simulink model "ADCS_FSM_test"  (R2025b)
settings: Solver=FixedStepDiscrete  StartTime=0.0  StopTime=10  FixedStep=0.1  RelTol=1e-3
settings Model: Creator=ADMIN  LastModifiedBy=ADMIN
settings DataIOCC: ExternalInput=ds  LoadExternalInput=on

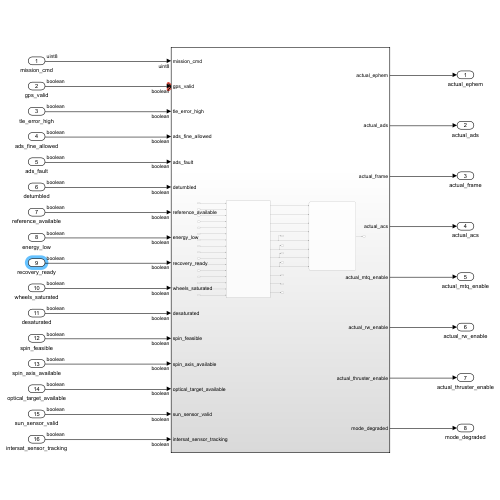
[thumbnail: Simulink's stored preview of the top-level diagram]
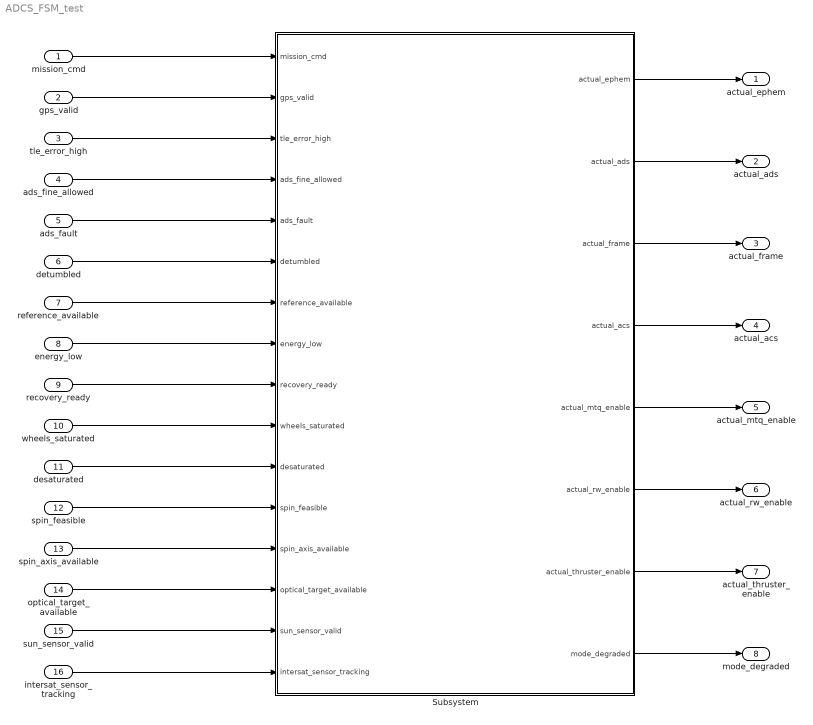
== system ADCS_FSM_test ==
  mission_cmd : Inport  OutDataTypeStr=uint8  PortDimensions=1
  gps_valid : Inport  Port=2  OutDataTypeStr=boolean  PortDimensions=1
  tle_error_high : Inport  Port=3  OutDataTypeStr=boolean  PortDimensions=1
  ads_fine_allowed : Inport  Port=4  OutDataTypeStr=boolean  PortDimensions=1
  ads_fault : Inport  Port=5  OutDataTypeStr=boolean  PortDimensions=1
  detumbled : Inport  Port=6  OutDataTypeStr=boolean  PortDimensions=1
  reference_available : Inport  Port=7  OutDataTypeStr=boolean  PortDimensions=1
  energy_low : Inport  Port=8  OutDataTypeStr=boolean  PortDimensions=1
  recovery_ready : Inport  Port=9  OutDataTypeStr=boolean  PortDimensions=1
  wheels_saturated : Inport  Port=10  OutDataTypeStr=boolean  PortDimensions=1
  desaturated : Inport  Port=11  OutDataTypeStr=boolean  PortDimensions=1
  spin_feasible : Inport  Port=12  OutDataTypeStr=boolean  PortDimensions=1
  spin_axis_available : Inport  Port=13  OutDataTypeStr=boolean  PortDimensions=1
  optical_target_available : Inport  Port=14  OutDataTypeStr=boolean  PortDimensions=1
  sun_sensor_valid : Inport  Port=15  OutDataTypeStr=boolean  PortDimensions=1
  intersat_sensor_tracking : Inport  Port=16  OutDataTypeStr=boolean  PortDimensions=1
  Subsystem : Subsystem
  actual_ephem : Outport
  actual_ads : Outport  Port=2
  actual_frame : Outport  Port=3
  actual_acs : Outport  Port=4
  actual_mtq_enable : Outport  Port=5
  actual_rw_enable : Outport  Port=6
  actual_thruster_enable : Outport  Port=7
  mode_degraded : Outport  Port=8
  wires:
  mission_cmd/1 -> Subsystem/1(mission_cmd)
  tle_error_high/1 -> Subsystem/3(tle_error_high)
  ads_fine_allowed/1 -> Subsystem/4(ads_fine_allowed)
  ads_fault/1 -> Subsystem/5(ads_fault)
  wheels_saturated/1 -> Subsystem/10(wheels_saturated)
  Subsystem/1(actual_ephem) -> actual_ephem/1
  Subsystem/8(mode_degraded) -> mode_degraded/1
  Subsystem/2(actual_ads) -> actual_ads/1
  Subsystem/3(actual_frame) -> actual_frame/1
  Subsystem/4(actual_acs) -> actual_acs/1
  Subsystem/5(actual_mtq_enable) -> actual_mtq_enable/1
  Subsystem/6(actual_rw_enable) -> actual_rw_enable/1
  Subsystem/7(actual_thruster_enable) -> actual_thruster_enable/1
  recovery_ready/1 -> Subsystem/9(recovery_ready)
  spin_feasible/1 -> Subsystem/12(spin_feasible)
  spin_axis_available/1 -> Subsystem/13(spin_axis_available)
  sun_sensor_valid/1 -> Subsystem/15(sun_sensor_valid)
  gps_valid/1 -> Subsystem/2(gps_valid)
  detumbled/1 -> Subsystem/6(detumbled)
  reference_available/1 -> Subsystem/7(reference_available)
  energy_low/1 -> Subsystem/8(energy_low)
  desaturated/1 -> Subsystem/11(desaturated)
  optical_target_available/1 -> Subsystem/14(optical_target_available)
  intersat_sensor_tracking/1 -> Subsystem/16(intersat_sensor_tracking)

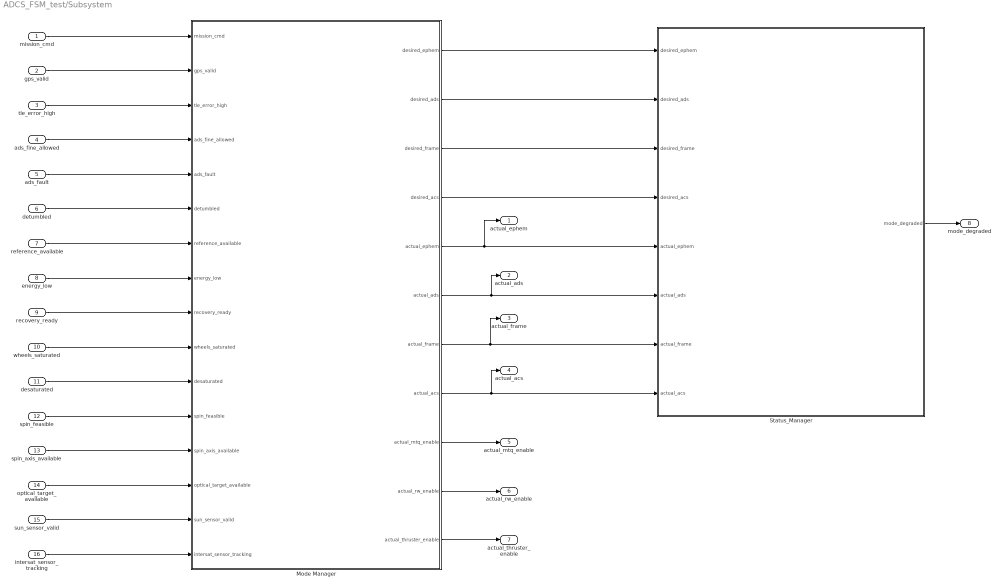
== system ADCS_FSM_test/Subsystem ==
  mission_cmd : Inport
  gps_valid : Inport  Port=2
  tle_error_high : Inport  Port=3
  ads_fine_allowed : Inport  Port=4
  ads_fault : Inport  Port=5
  detumbled : Inport  Port=6
  reference_available : Inport  Port=7
  energy_low : Inport  Port=8
  recovery_ready : Inport  Port=9
  wheels_saturated : Inport  Port=10
  desaturated : Inport  Port=11
  spin_feasible : Inport  Port=12
  spin_axis_available : Inport  Port=13
  optical_target_available : Inport  Port=14
  sun_sensor_valid : Inport  Port=15
  intersat_sensor_tracking : Inport  Port=16
  Mode Manager : Subsystem
  Status_Manager : Stateflow chart  TreatAsAtomicUnit=on
  actual_ephem : Outport
  actual_ads : Outport  Port=2
  actual_frame : Outport  Port=3
  actual_acs : Outport  Port=4
  actual_mtq_enable : Outport  Port=5
  actual_rw_enable : Outport  Port=6
  actual_thruster_enable : Outport  Port=7
  mode_degraded : Outport  Port=8
  wires:
  recovery_ready/1 -> Mode Manager/9(recovery_ready)
  Mode Manager/9(actual_mtq_enable) -> actual_mtq_enable/1
  Mode Manager/10(actual_rw_enable) -> actual_rw_enable/1
  Mode Manager/2(desired_ads) -> Status_Manager/2(desired_ads)
  Mode Manager/8(actual_acs) -> Status_Manager/8(actual_acs), actual_acs/1
  Mode Manager/1(desired_ephem) -> Status_Manager/1(desired_ephem)
  Mode Manager/5(actual_ephem) -> Status_Manager/5(actual_ephem), actual_ephem/1
  Mode Manager/6(actual_ads) -> Status_Manager/6(actual_ads), actual_ads/1
  Mode Manager/7(actual_frame) -> Status_Manager/7(actual_frame), actual_frame/1
  Mode Manager/3(desired_frame) -> Status_Manager/3(desired_frame)
  Mode Manager/4(desired_acs) -> Status_Manager/4(desired_acs)
  reference_available/1 -> Mode Manager/7(reference_available)
  mission_cmd/1 -> Mode Manager/1(mission_cmd)
  ads_fault/1 -> Mode Manager/5(ads_fault)
  ads_fine_allowed/1 -> Mode Manager/4(ads_fine_allowed)
  Mode Manager/11(actual_thruster_enable) -> actual_thruster_enable/1
  wheels_saturated/1 -> Mode Manager/10(wheels_saturated)
  optical_target_available/1 -> Mode Manager/14(optical_target_available)
  detumbled/1 -> Mode Manager/6(detumbled)
  intersat_sensor_tracking/1 -> Mode Manager/16(intersat_sensor_tracking)
  desaturated/1 -> Mode Manager/11(desaturated)
  spin_feasible/1 -> Mode Manager/12(spin_feasible)
  tle_error_high/1 -> Mode Manager/3(tle_error_high)
  energy_low/1 -> Mode Manager/8(energy_low)
  Status_Manager/1(mode_degraded) -> mode_degraded/1
  spin_axis_available/1 -> Mode Manager/13(spin_axis_available)
  sun_sensor_valid/1 -> Mode Manager/15(sun_sensor_valid)
  gps_valid/1 -> Mode Manager/2(gps_valid)

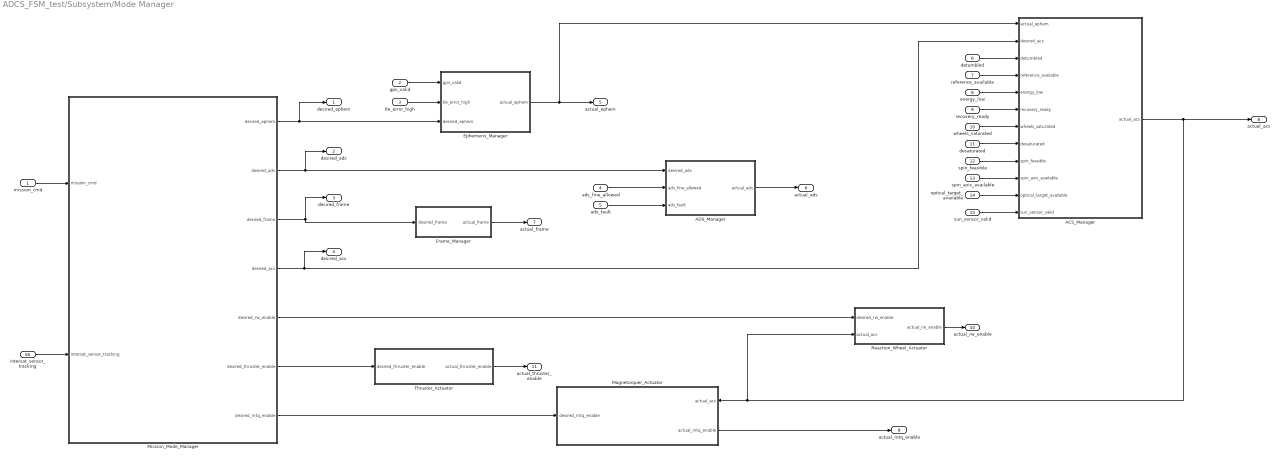
== system ADCS_FSM_test/Subsystem/Mode Manager ==
  mission_cmd : Inport  OutDataTypeStr=uint8  PortDimensions=1
  gps_valid : Inport  Port=2  OutDataTypeStr=boolean  PortDimensions=1
  tle_error_high : Inport  Port=3  OutDataTypeStr=boolean  PortDimensions=1
  ads_fine_allowed : Inport  Port=4  OutDataTypeStr=boolean  PortDimensions=1
  ads_fault : Inport  Port=5  OutDataTypeStr=boolean  PortDimensions=1
  detumbled : Inport  Port=6  OutDataTypeStr=boolean  PortDimensions=1
  reference_available : Inport  Port=7  OutDataTypeStr=boolean  PortDimensions=1
  energy_low : Inport  Port=8  OutDataTypeStr=boolean  PortDimensions=1
  recovery_ready : Inport  Port=9  OutDataTypeStr=boolean  PortDimensions=1
  wheels_saturated : Inport  Port=10  OutDataTypeStr=boolean  PortDimensions=1
  desaturated : Inport  Port=11  OutDataTypeStr=boolean  PortDimensions=1
  spin_feasible : Inport  Port=12  OutDataTypeStr=boolean  PortDimensions=1
  spin_axis_available : Inport  Port=13  OutDataTypeStr=boolean  PortDimensions=1
  optical_target_available : Inport  Port=14  OutDataTypeStr=boolean  PortDimensions=1
  sun_sensor_valid : Inport  Port=15  OutDataTypeStr=boolean  PortDimensions=1
  intersat_sensor_tracking : Inport  Port=16  OutDataTypeStr=boolean  PortDimensions=1
  ACS_Manager : Stateflow chart  TreatAsAtomicUnit=on
      settings: PortSchema="{\"entries\":[{\"content\":{\"sides\":[{\"content\":{\"connectorIds\":[\"In2\",\"In1\",\"In3\",\"In4\",\"In5\",\"In6\",\"In7\",\"In8\",\"In9\",\"In10\",\"In11\",\"In12\"]},\"type\":\"ConnectorPlacement.EquallySpacedRectSide\",\"uuid\":\"c64f5ed7-7a07-4761-a251-d625087249f8\"},{\"content\":{\"connectorIds\":[\"Out1\"],\"side\":\"RIGHT\"},\"type\":\"ConnectorPlacement.EquallySpacedRectSide\",\"uuid\":\"ff17dfa7-5a32-4799-bec0-131df3b46d45\"},{\"content\":{\"side\":\"TOP\"},\"type\":\"ConnectorPlacement.EquallySpacedRectSide\",\"uuid\":\"acaf274e-12ec-4fab-ab7e-ad580afcef6e\"}]},\"type\":\"ConnectorPlacement.EquallySpacedConnector\",\"uuid\":\"7d19de63-b993-417e-b6e9-9dc888da130b\"}],\"packageUris\":[\"http://schema.mathworks.com/mf0/Connector/R2020b\"],\"version\":\"1.0\"}"
  ADS_Manager : Stateflow chart  TreatAsAtomicUnit=on
  Ephemeris_Manager : Stateflow chart  TreatAsAtomicUnit=on
      settings: PortSchema="{\"entries\":[{\"content\":{\"sides\":[{\"content\":{\"connectorIds\":[\"In2\",\"In3\",\"In1\"]},\"type\":\"ConnectorPlacement.EquallySpacedRectSide\",\"uuid\":\"cbbccf67-8c60-498d-a98a-76db8747fb3a\"},{\"content\":{\"connectorIds\":[\"Out1\"],\"side\":\"RIGHT\"},\"type\":\"ConnectorPlacement.EquallySpacedRectSide\",\"uuid\":\"743b35d2-d398-4833-9c20-93b5e77612f2\"},{\"content\":{\"side\":\"TOP\"},\"type\":\"ConnectorPlacement.EquallySpacedRectSide\",\"uuid\":\"56075cc1-c683-438a-85bf-78d94186ffa6\"}]},\"type\":\"ConnectorPlacement.EquallySpacedConnector\",\"uuid\":\"bae867d4-09fc-4097-a23b-eff5fb3633ac\"}],\"packageUris\":[\"http://schema.mathworks.com/mf0/Connector/R2020b\"],\"version\":\"1.0\"}"
  Frame_Manager : Stateflow chart  TreatAsAtomicUnit=on
  Magnetorquer_Actuator : Stateflow chart  TreatAsAtomicUnit=on
      settings: PortSchema="{\"entries\":[{\"content\":{\"sides\":[{\"content\":{\"connectorIds\":[\"In1\"]},\"type\":\"ConnectorPlacement.EquallySpacedRectSide\",\"uuid\":\"426f70af-d698-41ea-b496-30ad3acec41c\"},{\"content\":{\"connectorIds\":[\"In2\",\"Out1\"],\"side\":\"RIGHT\"},\"type\":\"ConnectorPlacement.EquallySpacedRectSide\",\"uuid\":\"1114bad5-09d2-4629-8a88-a540db9f7764\"},{\"content\":{\"side\":\"TOP\"},\"type\":\"ConnectorPlacement.EquallySpacedRectSide\",\"uuid\":\"f84a890c-1c78-4114-bb57-a5d0fdcf0e8c\"},{\"content\":{\"side\":\"BOTTOM\"},\"type\":\"ConnectorPlacement.EquallySpacedRectSide\",\"uuid\":\"d531b03e-0cd9-4f84-84e8-924ccdcb0c16\"}]},\"type\":\"ConnectorPlacement.EquallySpacedConnector\",\"uuid\":\"89862218-98b1-4fe4-8a9d-653868ce345b\"}],\"packageUris\":[\"http://schema.mathworks.com/mf0/Connector/R2020b\"],\"version\":\"1.0\"}"
  Mission_Mode_Manager : Stateflow chart  TreatAsAtomicUnit=on
      settings: PortSchema="{\"entries\":[{\"content\":{\"sides\":[{\"content\":{\"connectorIds\":[\"In1\",\"In2\"]},\"type\":\"ConnectorPlacement.EquallySpacedRectSide\",\"uuid\":\"e384235c-f18f-4250-9d30-176d1cc8fe20\"},{\"content\":{\"connectorIds\":[\"Out1\",\"Out2\",\"Out3\",\"Out4\",\"Out6\",\"Out7\",\"Out5\"],\"side\":\"RIGHT\"},\"type\":\"ConnectorPlacement.EquallySpacedRectSide\",\"uuid\":\"96497599-ce3f-49ba-a8c7-fe298164a70d\"},{\"content\":{\"side\":\"TOP\"},\"type\":\"ConnectorPlacement.EquallySpacedRectSide\",\"uuid\":\"b5d3b03c-2d36-4a59-acbf-0bb54c486367\"},{\"content\":{\"side\":\"BOTTOM\"},\"type\":\"ConnectorPlacement.EquallySpacedRectSide\",\"uuid\":\"daf0fe9a-2cb8-4f81-925b-bbc871b2e354\"}]},\"type\":\"ConnectorPlacement.EquallySpacedConnector\",\"uuid\":\"8f1f8c95-3de9-4666-afa6-9b16d5d2b405\"}],\"packageUris\":[\"http://schema.mathworks.com/mf0/Connector/R2020b\"],\"version\":\"1.0\"}"
  Reaction_Wheel_Actuator : Stateflow chart  TreatAsAtomicUnit=on
  Thruster_Actuator : Stateflow chart  TreatAsAtomicUnit=on
  desired_ephem : Outport
  desired_ads : Outport  Port=2
  desired_frame : Outport  Port=3
  desired_acs : Outport  Port=4
  actual_ephem : Outport  Port=5
  actual_ads : Outport  Port=6
  actual_frame : Outport  Port=7
  actual_acs : Outport  Port=8
  actual_mtq_enable : Outport  Port=9
  actual_rw_enable : Outport  Port=10
  actual_thruster_enable : Outport  Port=11
  wires:
  sun_sensor_valid/1 -> ACS_Manager/12(sun_sensor_valid)
  ACS_Manager/1(actual_acs) -> actual_acs/1, Magnetorquer_Actuator/2(actual_acs), Reaction_Wheel_Actuator/2(actual_acs)
  Mission_Mode_Manager/4(desired_acs) -> desired_acs/1, ACS_Manager/1(desired_acs)
  Mission_Mode_Manager/6(desired_rw_enable) -> Reaction_Wheel_Actuator/1(desired_rw_enable)
  energy_low/1 -> ACS_Manager/5(energy_low)
  Magnetorquer_Actuator/1(actual_mtq_enable) -> actual_mtq_enable/1
  Mission_Mode_Manager/5(desired_mtq_enable) -> Magnetorquer_Actuator/1(desired_mtq_enable)
  Mission_Mode_Manager/1(desired_ephem) -> desired_ephem/1, Ephemeris_Manager/1(desired_ephem)
  Frame_Manager/1(actual_frame) -> actual_frame/1
  optical_target_available/1 -> ACS_Manager/11(optical_target_available)
  Mission_Mode_Manager/2(desired_ads) -> desired_ads/1, ADS_Manager/1(desired_ads)
  tle_error_high/1 -> Ephemeris_Manager/3(tle_error_high)
  reference_available/1 -> ACS_Manager/4(reference_available)
  detumbled/1 -> ACS_Manager/3(detumbled)
  Mission_Mode_Manager/7(desired_thruster_enable) -> Thruster_Actuator/1(desired_thruster_enable)
  wheels_saturated/1 -> ACS_Manager/7(wheels_saturated)
  Mission_Mode_Manager/3(desired_frame) -> desired_frame/1, Frame_Manager/1(desired_frame)
  ADS_Manager/1(actual_ads) -> actual_ads/1
  Reaction_Wheel_Actuator/1(actual_rw_enable) -> actual_rw_enable/1
  ads_fine_allowed/1 -> ADS_Manager/2(ads_fine_allowed)
  Ephemeris_Manager/1(actual_ephem) -> ACS_Manager/2(actual_ephem), actual_ephem/1
  gps_valid/1 -> Ephemeris_Manager/2(gps_valid)
  intersat_sensor_tracking/1 -> Mission_Mode_Manager/2(intersat_sensor_tracking)
  ads_fault/1 -> ADS_Manager/3(ads_fault)
  recovery_ready/1 -> ACS_Manager/6(recovery_ready)
  Thruster_Actuator/1(actual_thruster_enable) -> actual_thruster_enable/1
  mission_cmd/1 -> Mission_Mode_Manager/1(mission_cmd)
  spin_axis_available/1 -> ACS_Manager/10(spin_axis_available)
  desaturated/1 -> ACS_Manager/8(desaturated)
  spin_feasible/1 -> ACS_Manager/9(spin_feasible)

== stateflow chart ADCS_FSM_test/Subsystem/Mode Manager/Frame_Manager ==
  state FRAME_INERTIAL
    entry:
    actual_frame = uint8(2);
  state FRAME_LVLH
    entry:
    actual_frame = uint8(3);
  state FRAME_BODY
    entry:
    actual_frame = uint8(1);
  state FRAME_EARTH_TARGET
    entry:
    actual_frame = uint8(4);
  state FRAME_IDLE
    entry:
    actual_frame = uint8(0);
  state FRAME_IMAGING_TDI
    entry:
    actual_frame = uint8(6);
  state FRAME_VNB
    entry:
    actual_frame = uint8(5);
  FRAME_INERTIAL -> (junction 11) : [desired_frame ~= uint8(2)]
  (junction 11) -> FRAME_INERTIAL [order 3] : [desired_frame == uint8(2)]
  FRAME_LVLH -> (junction 11) : [desired_frame ~= uint8(3)]
  (junction 11) -> FRAME_LVLH [order 4] : [desired_frame == uint8(3)]
  FRAME_BODY -> (junction 11) : [desired_frame ~= uint8(1)]
  (junction 11) -> FRAME_BODY [order 2] : [desired_frame == uint8(1)]
  FRAME_EARTH_TARGET -> (junction 11) : [desired_frame ~= uint8(4)]
  (junction 11) -> FRAME_EARTH_TARGET [order 5] : [desired_frame == uint8(4)]
  (junction 11) -> FRAME_IDLE [order 1] : [desired_frame == uint8(0)]
  FRAME_IDLE -> (junction 11) : [desired_frame ~= uint8(0)]
  FRAME_IMAGING_TDI -> (junction 11) : [desired_frame ~= uint8(6)]
  (junction 11) -> FRAME_VNB [order 6] : [desired_frame == uint8(5)]
  (junction 11) -> FRAME_IMAGING_TDI [order 7] : [desired_frame == uint8(6)]
  FRAME_VNB -> (junction 11) : [desired_frame ~= uint8(5)]
  (default) -> FRAME_IDLE
  data: desired_frame input uint8; actual_frame output uint8 =0

== stateflow chart ADCS_FSM_test/Subsystem/Mode Manager/ACS_Manager ==
  state ACS_DETUMBLE
    entry:
    actual_acs = uint8(1);
  state ACS_POINT
    entry:
    actual_acs = uint8(2);
  state ACS_IDLE
    entry:
    actual_acs = uint8(0);
  state ACS_SLEW_SLOW
    entry:
    actual_acs = uint8(4);
  state ACS_DESAT
    entry:
    actual_acs = uint8(7);
    %exit:
    %desaturated = 1;
  state ACS_HOLD
    entry:
    actual_acs = uint8(3);
  state ACS_OPTICAL
    entry:
    actual_acs = uint8(8);
  state ACS_SPIN
    entry:
    actual_acs = uint8(6);
  state ACS_SLEW_FAST
    entry:
    actual_acs = uint8(5);
  state ACS_SAFE
    entry:
    actual_acs = uint8(9);
  ACS_SLEW_SLOW -> ACS_DESAT [order 3] : [wheels_saturated && ~energy_low]
  ACS_OPTICAL -> ACS_POINT [order 3] : [~optical_target_available &&...
      |  ~energy_low]
  (junction 25) -> ACS_DETUMBLE [order 2] : [desired_acs == uint8(1)]
  ACS_DETUMBLE -> (junction 25) : [desired_acs ~= uint8(1)]
  ACS_POINT -> ACS_SAFE [order 2] : [energy_low || ~reference_available ||...
      |  ~detumbled || actual_ephem == uint8(0)]
  (junction 25) -> ACS_IDLE [order 1] : [desired_acs == uint8(0)]
  ACS_POINT -> (junction 25) [order 1] : [desired_acs ~= uint8(2) &&...
      |  ~(desired_acs == uint8(8) &&...
      |  ~optical_target_available)]
  (junction 25) -> ACS_POINT [order 3] : [desired_acs == uint8(2)]
  (default) -> ACS_IDLE
  ACS_IDLE -> (junction 25) : [desired_acs ~= uint8(0)]
  (junction 25) -> ACS_SLEW_SLOW [order 5] : [desired_acs == uint8(4)]
  ACS_SLEW_SLOW -> (junction 25) [order 1] : [desired_acs ~= uint8(4)]
  ACS_SLEW_SLOW -> ACS_SAFE [order 2] : [energy_low || ~detumbled ||...
      |  actual_ephem == uint8(0)]
  ACS_HOLD -> (junction 25) [order 1] : [desired_acs ~= uint8(3)]
  ACS_DESAT -> (junction 25) [order 1] : [desired_acs ~= uint8(7) &&...
      |  desaturated && recovery_ready &&...
      |  ~energy_low]
  (junction 25) -> ACS_HOLD [order 4] : [desired_acs == uint8(3)]
  (junction 25) -> ACS_DESAT [order 8] : [desired_acs == uint8(7)]
  ACS_OPTICAL -> (junction 25) [order 1] : [desired_acs ~= uint8(8) && optical_target_available]
  (junction 25) -> ACS_OPTICAL [order 9] : [desired_acs == uint8(8)]
  (junction 25) -> ACS_SLEW_FAST [order 6] : [desired_acs == uint8(5)]
  ACS_SLEW_FAST -> (junction 25) [order 1] : [desired_acs ~= uint8(5)]
  ACS_SAFE -> (junction 25) : [desired_acs ~= uint8(9) &&...
      |  ~energy_low && recovery_ready &&...
      |  sun_sensor_valid && ~((desired_acs == uint8(2)) &&...
      |  ~reference_available) && ~((desired_acs == uint8(6)) &&...
      |  (~spin_feasible || ~spin_axis_available))]
  (junction 25) -> ACS_SAFE [order 10] : [desired_acs == uint8(9)]
  (junction 25) -> ACS_SPIN [order 7] : [desired_acs == uint8(6)]
  ACS_SPIN -> (junction 25) [order 2] : [desired_acs ~= uint8(6)]
  ACS_DESAT -> ACS_SAFE [order 2] : [energy_low]
  ACS_SLEW_FAST -> ACS_DESAT [order 3] : [wheels_saturated && ~energy_low]
  ACS_HOLD -> ACS_SAFE [order 2] : [energy_low ||...
      |  ~detumbled ||...
      |  actual_ephem == uint8(0)]
  ACS_OPTICAL -> ACS_SAFE [order 2] : [energy_low]
  ACS_SPIN -> ACS_SAFE [order 1] : [energy_low || ~spin_feasible ||...
      |  ~spin_axis_available]
  ACS_SLEW_FAST -> ACS_SAFE [order 2] : [energy_low || ~detumbled ||...
      |  actual_ephem == uint8(0)]
  data: desired_acs input uint8; actual_ephem input uint8; detumbled input boolean; reference_available input boolean; energy_low input boolean; recovery_ready input boolean; wheels_saturated input boolean; desaturated input boolean; spin_feasible input boolean; spin_axis_available input boolean; optical_target_available input boolean; sun_sensor_valid input boolean; actual_acs output uint8 =0

== stateflow chart ADCS_FSM_test/Subsystem/Mode Manager/Magnetorquer_Actuator ==
  state OFF
    entry:
    actual_mtq_enable = false;
  state ON
    entry:
    actual_mtq_enable = true;
  ON -> OFF : [~(desired_mtq_enable || actual_acs == uint8(7))]
  (default) -> OFF
  OFF -> ON : [desired_mtq_enable || actual_acs == uint8(7)]
  data: desired_mtq_enable input boolean; actual_acs input uint8; actual_mtq_enable output boolean =0

== stateflow chart ADCS_FSM_test/Subsystem/Mode Manager/Reaction_Wheel_Actuator ==
  state OFF
    entry:
    actual_rw_enable = false;
  state ON
    entry:
    actual_rw_enable = true;
  ON -> OFF : [~(desired_rw_enable && actual_acs ~= uint8(7))]
  OFF -> ON : [desired_rw_enable && actual_acs ~= uint8(7)]
  (default) -> OFF
  data: desired_rw_enable input boolean; actual_acs input uint8; actual_rw_enable output boolean =0

== stateflow chart ADCS_FSM_test/Subsystem/Mode Manager/Thruster_Actuator ==
  state OFF
    entry:
    actual_thruster_enable = false;
  state ON
    entry:
    actual_thruster_enable = true;
  ON -> OFF : [~(desired_thruster_enable)]
  OFF -> ON : [desired_thruster_enable]
  (default) -> OFF
  data: desired_thruster_enable input boolean; actual_thruster_enable output boolean =0

== stateflow chart ADCS_FSM_test/Subsystem/Status_Manager ==
  state STATUS
    during:
    mode_degraded = (actual_ephem ~= desired_ephem) || (actual_ads ~= desired_ads) || (actual_frame ~= desired_frame) || (actual_acs ~= desired_acs);
  (default) -> STATUS
  data: desired_ephem input uint8; desired_ads input uint8; desired_frame input uint8; desired_acs input uint8; actual_ephem input uint8; actual_ads input uint8; actual_frame input uint8; actual_acs input uint8; mode_degraded output boolean =0

== stateflow chart ADCS_FSM_test/Subsystem/Mode Manager/Ephemeris_Manager ==
  state EPHEM_IDLE
    entry:
    actual_ephem = uint8(0);
  state EPHEM_GPS
    entry:
    actual_ephem = uint8(2);
  state EPHEM_TLE
    entry:
    actual_ephem = uint8(1);
  EPHEM_GPS -> EPHEM_IDLE [order 1] : [desired_ephem == uint8(0)]
  EPHEM_IDLE -> EPHEM_GPS [order 2] : [desired_ephem == uint8(2)...
      |  && gps_valid]
  (default) -> EPHEM_IDLE
  EPHEM_IDLE -> EPHEM_TLE [order 1] : [desired_ephem == uint8(1) ||...
      |  (desired_ephem == uint8(2) &&...
      |  ~gps_valid && ~tle_error_high)]
  EPHEM_TLE -> EPHEM_IDLE [order 1] : [desired_ephem == uint8(0)...
      |  || tle_error_high]
  EPHEM_GPS -> EPHEM_TLE [order 2] : [desired_ephem == uint8(1) ||...
      |  ~gps_valid]
  EPHEM_TLE -> EPHEM_GPS [order 2] : [desired_ephem == uint8(2) && gps_valid]
  data: desired_ephem input uint8; gps_valid input boolean; tle_error_high input boolean; actual_ephem output uint8 =0

== stateflow chart ADCS_FSM_test/Subsystem/Mode Manager/ADS_Manager ==
  state ADS_IDLE
    entry:
    actual_ads = uint8(0);
  state ADS_UKF_FINE
    entry:
    actual_ads = uint8(2);
  state ADS_UKF_COARSE
    entry:
    actual_ads = uint8(1);
  ADS_UKF_FINE -> ADS_IDLE [order 2] : [desired_ads == uint8(0) || ads_fault]
  ADS_IDLE -> ADS_UKF_FINE [order 2] : [desired_ads == uint8(2) &&...
      |  ads_fine_allowed && ~ads_fault]
  (default) -> ADS_IDLE
  ADS_UKF_COARSE -> ADS_IDLE [order 1] : [desired_ads == uint8(0) || ads_fault]
  ADS_IDLE -> ADS_UKF_COARSE [order 1] : [desired_ads == uint8(1) ||...
      |  (desired_ads == uint8(2) &&...
      |  ~ads_fine_allowed)]
  ADS_UKF_FINE -> ADS_UKF_COARSE [order 1] : [desired_ads == uint8(1) ||...
      |  ~ads_fine_allowed]
  ADS_UKF_COARSE -> ADS_UKF_FINE [order 2] : [desired_ads == uint8(2) &&...
      |  ads_fine_allowed && ~ads_fault]
  data: desired_ads input uint8; ads_fine_allowed input boolean; ads_fault input boolean; actual_ads output uint8 =0

== stateflow chart ADCS_FSM_test/Subsystem/Mode Manager/Mission_Mode_Manager ==
  state M_DETUMBLE
    entry:
    desired_ephem = uint8(0);
    desired_ads = uint8(1);
    desired_frame = uint8(0);
    desired_acs = uint8(1);
    desired_mtq_enable = true;
    desired_rw_enable = false;
    desired_thruster_enable = true;
  state M_SAFE_SUN
    entry:
    desired_ephem = uint8(0);
    desired_ads = uint8(0);
    desired_frame = uint8(0);
    desired_acs = uint8(9);
    desired_mtq_enable = false;
    desired_rw_enable = true;
    desired_thruster_enable = false;
  state M_Y_SPIN
    entry:
    desired_ephem = uint8(2);
    desired_ads = uint8(1);
    desired_frame = uint8(3);
    desired_acs = uint8(6);
    desired_mtq_enable = false;
    desired_rw_enable = true;
    desired_thruster_enable = false;
    % desired_thruster_enable = ~spin_feasible;
  state M_IDLE
    entry:
    desired_ephem = uint8(0);
    desired_ads = uint8(0);
    desired_frame = uint8(0);
    desired_acs = uint8(0);
    desired_mtq_enable = false;
    desired_rw_enable = false;
    desired_thruster_enable = false;
  state M_MINMAX_DRAG
    entry:
    desired_ephem = uint8(2);
    desired_ads = uint8(2);
    desired_frame = uint8(3);
    %desired_frame = uint8(3 + 2 * drag_use_vnb);
    desired_acs = uint8(2);
    desired_mtq_enable = false;
    desired_rw_enable = true;
    desired_thruster_enable = false;
  state M_POINT_NADIR
    entry:
    desired_ephem = uint8(2);
    desired_ads = uint8(2);
    desired_frame = uint8(3);
    desired_acs = uint8(2);
    desired_mtq_enable = false;
    desired_rw_enable = true;
    desired_thruster_enable = false;
  state M_SLEW_FIXED
    entry:
    desired_ephem = uint8(2);
    desired_ads = uint8(2);
    desired_frame = uint8(2);
    desired_acs = uint8(4);
    desired_mtq_enable = false;
    desired_rw_enable = true;
    desired_thruster_enable = false;
    % desired_thruster_enable = ~slew_feasible;
  state M_SLEW_FASTEST
    entry:
    desired_ephem = uint8(2);
    desired_ads = uint8(2);
    desired_frame = uint8(2);
    desired_acs = uint8(5);
    desired_mtq_enable = false;
    desired_rw_enable = true;
    desired_thruster_enable = false;
  state M_POINT_MOON
    entry:
    desired_ephem = uint8(2);
    desired_ads = uint8(2);
    desired_frame = uint8(2);
    desired_acs = uint8(2);
    desired_mtq_enable = false;
    desired_rw_enable = true;
    desired_thruster_enable = false;
  state M_TDI
    entry:
    desired_ephem = uint8(2);
    desired_ads = uint8(2);
    desired_frame = uint8(6);
    desired_acs = uint8(2);
    desired_mtq_enable = false;
    desired_rw_enable = true;
    desired_thruster_enable = false;
  state M_POINT_SUN
    entry:
    desired_ephem = uint8(2);
    desired_ads = uint8(2);
    desired_frame = uint8(2);
    desired_acs = uint8(3);
    desired_mtq_enable = false;
    desired_rw_enable = true;
    desired_thruster_enable = false;
  state M_INTERSAT_TRACK
    entry:
    desired_ephem = uint8(2);
    desired_ads = uint8(2);
    desired_frame = uint8(2);
    desired_acs = uint8(2 + 6 * intersat_sensor_tracking);
    desired_mtq_enable = false;
    desired_rw_enable = true;
    desired_thruster_enable = false;
  M_DETUMBLE -> (junction 28) : [mission_cmd ~= uint8(1)]
  (junction 28) -> M_DETUMBLE [order 2] : [mission_cmd == uint8(1)]
  M_Y_SPIN -> (junction 28) : [mission_cmd ~= uint8(3)]
  M_SAFE_SUN -> (junction 28) : [mission_cmd ~= uint8(2)]
  (junction 28) -> M_SAFE_SUN [order 3] : [mission_cmd == uint8(2)]
  M_IDLE -> (junction 28) : [mission_cmd ~= uint8(0)]
  (default) -> M_IDLE
  (junction 28) -> M_IDLE [order 1] : [mission_cmd == uint8(0)]
  (junction 28) -> M_Y_SPIN [order 4] : [mission_cmd == uint8(3)]
  (junction 28) -> M_MINMAX_DRAG [order 12] : [mission_cmd == uint8(11)]
  M_MINMAX_DRAG -> (junction 28) : [mission_cmd ~= uint8(11)]
  (junction 28) -> M_POINT_NADIR [order 5] : [mission_cmd == uint8(4)]
  M_POINT_NADIR -> (junction 28) : [mission_cmd ~= uint8(4)]
  (junction 28) -> M_SLEW_FIXED [order 8] : [mission_cmd == uint8(7)]
  M_SLEW_FASTEST -> (junction 28) : [mission_cmd ~= uint8(8)]
  (junction 28) -> M_SLEW_FASTEST [order 9] : [mission_cmd == uint8(8)]
  M_SLEW_FIXED -> (junction 28) : [mission_cmd ~= uint8(7)]
  (junction 28) -> M_POINT_MOON [order 7] : [mission_cmd == uint8(6)]
  (junction 28) -> M_POINT_SUN [order 6] : [mission_cmd == uint8(5)]
  M_POINT_MOON -> (junction 28) : [mission_cmd ~= uint8(6)]
  M_POINT_SUN -> (junction 28) : [mission_cmd ~= uint8(5)]
  (junction 28) -> M_INTERSAT_TRACK [order 10] : [mission_cmd == uint8(9)]
  (junction 28) -> M_TDI [order 11] : [mission_cmd == uint8(10)]
  M_INTERSAT_TRACK -> (junction 28) : [mission_cmd ~= uint8(9)]
  M_TDI -> (junction 28) : [mission_cmd ~= uint8(10)]
  data: mission_cmd input uint8; intersat_sensor_tracking input boolean; desired_ephem output uint8 =0; desired_ads output uint8 =0; desired_frame output uint8 =0; desired_acs output uint8 =0; desired_mtq_enable output boolean =0; desired_rw_enable output boolean =0; desired_thruster_enable output boolean =0
